simulink model "gtm_design"  (R2021b)
settings: Solver=VariableStepAuto  StartTime=0.0  StopTime=10.0  MinStep=0.00999  RelTol=1e-3
StopFcn:
  | MWSout=grabmws(bdroot);
  | MWSout.lastrun=datestr(now);
values from neighbouring files (symbols this model uses):
  knots2fps = 1.68781    [setup.m]
  s = tf('s')    [setup.m]
undefined symbols (not defined in the file or in its folder): Aero, aftfuel, aftfuel_pos, AILL, AILLC, AILR, AILRC, alpha_deg, alt0, altitude_ft, Ax_g, Ay_g, Az_g, b, beta_deg, bias, BRAKEC, Cbar, cg_pos0, cg_shift_gear, ControlMode, DamageCase, DamageModels, DamageOnsetTime, deltc, Earth, ELLIB, ELLIBC, ELLOB, ELLOBC, ELRIB, ELRIBC, ELROB, ELROBC, engl_ang, engl_pos, engr_ang, engr_pos, etas0, etas1, etasc_feedthrough, FLAPLC, FLAPLIB, FLAPLOB, FLAPRC, FLAPRIB, FLAPROB, FlightMode, FuelUsed_Init, fwdfuel, fwdfuel_pos, GEAR, GEARC, Inertia0, Inertia_shift_gear, Ixx_model, Iyy_model, Izz_model, KTAS, LandingGear ... (+66)
libraries: simulink_extras x98, LPVBlockLibrary x54, simulink_need_slupdate x30, aerolibconvert2 x27, simulink x7, aerolibtransform2 x6, uavalgslib x4, UserContent_lib x2, robotcorelib x1, uavutilslib x1
(part 4 of 9)

== system gtm_design/GTM_T2/Engines/Right_Engine Jetcat P70 ==
  Throttle : Inport
  pratio : Inport  Port=2
  tratio : Inport  Port=3
  BypassDynamics : Inport  Port=4
  qbar : Inport  Port=5
  S : Inport  Port=6
  Fuel Pump Voltage : Lookup  InputValues=fuelflow_table  Table=fuelpump_table  LookUpMeth=Interpolation-Use End Values
  Product2 : Product  RndMeth=Zero
  RPMref_2_EGT : Polyval  Coefs=Coeff_EGT
  RPMref_2_FuelFlow : Polyval  Coefs=Coeff_fuelflow
  RPMref_2_Thrust : Polyval  Coefs=Coeff_thrust
  Saturation : Saturate  UpperLimit=inf  LowerLimit=0
  Simple Ram Drag Model : MATLAB Function  TreatAsAtomicUnit=on
  Sum : Sum  Inputs=-+|
  Switch : Switch  Criteria=u2 ~= 0
  Terminator : Terminator
  Throttle Lag1 : Subsystem
  Throttle2 : InportShadow
  Throttle_2_RPMref : Polyval  Coefs=Coeff_throttle
  UnScale_Ref_RPM : Gain  Gain=123000/100
  angular momentum : Gain  Gain=(pi*shaft_dia^4/32) * shaft_len * density * (2*pi/60)
  Thrust (lbf) : Outport
  RPM : Outport  Port=2
  h (slg-ft^2/s) : Outport  Port=3
  Fuel Pump Voltage (V) : Outport  Port=4
  EGT (deg C) : Outport  Port=5
  Fuel Flow (lbs/min) : Outport  Port=6
  wires:
  Saturation/1 -> Thrust (lbf)/1
  Sum/1 -> Saturation/1
  Product2/1 -> Sum/2
  Simple Ram Drag Model/1(ram_drag) -> Sum/1
  S/1 -> Simple Ram Drag Model/2(S)
  qbar/1 -> Simple Ram Drag Model/1(qbar)
  Throttle2/1 -> Switch/1
  BypassDynamics/1 -> Switch/2
  Throttle Lag1/1(y) -> Switch/3  "Throttle_Lag"
  Switch/1 -> Throttle_2_RPMref/1
  Throttle/1 -> Throttle Lag1/1(throttle)
  Throttle_2_RPMref/1 -> RPMref_2_Thrust/1, UnScale_Ref_RPM/1, RPMref_2_EGT/1, RPMref_2_FuelFlow/1
  angular momentum/1 -> h (slg-ft^2/s)/1
  UnScale_Ref_RPM/1 -> angular momentum/1, RPM/1
  tratio/1 -> Terminator/1
  RPMref_2_Thrust/1 -> Product2/1
  RPMref_2_FuelFlow/1 -> Fuel Flow (lbs/min)/1, Fuel Pump Voltage/1
  pratio/1 -> Product2/2
  Fuel Pump Voltage/1 -> Fuel Pump Voltage (V)/1
  RPMref_2_EGT/1 -> EGT (deg C)/1

== system gtm_design/GTM_T2/Landing Gear/LandingGear ==
  cg : Inport  PortDimensions=3
  EulerAngles (Rad) : Inport  Port=2  PortDimensions=3
  Altitude (ft) : Inport  Port=3  PortDimensions=1
  pqr (Rad/sec) : Inport  Port=4  PortDimensions=3
  Vbody (ft/sec) : Inport  Port=5  PortDimensions=3
  Heading (Rad) : Inport  Port=6  PortDimensions=1
  Brake (0-1) : Inport  Port=7  PortDimensions=1
  Steer (deg) : Inport  Port=8  PortDimensions=1
  geardown (0/1) : Inport  Port=9  PortDimensions=1
  Data Type Conversion : DataTypeConversion  OutDataTypeStr=int32
  Euler to DCM1 : Subsystem
  Math Function : Math  Operator=transpose  SignedPower=on  SaturateOnIntegerOverflow=on
  Math Function1 : Math  Operator=transpose  SignedPower=on  SaturateOnIntegerOverflow=on
  Product : Product  Multiplication=Matrix(*)  RndMeth=Zero
  Reshape : Reshape
  S-Function1 : S-Function  FunctionName=gear_sfcn  SFunctionDeploymentMode=off  EnableBusSupport=off
  Subsystem : Subsystem
  Wheel Positions : Constant  Value=[NoseWheelPos(:);LeftMainPos(:); RightMainPos(:)];
  Wheel Positions1 : Constant  Value=SpringConst
  Wheel Positions2 : Constant  Value=DampingConst
  Wheel Positions3 : Constant  Value=MountStiffness
  Wheel Positions4 : Constant  Value=StrokeLength
  Wheel Positions5 : Constant  Value=MountDamping
  F_gear : Outport
  M_gear : Outport  Port=2
  Contact : Outport  Port=3
  wires:
  Wheel Positions5/1 -> S-Function1/5
  Math Function1/1 -> Product/1
  Vbody (ft/sec)/1 -> Product/2
  Euler to DCM1/1(DCM) -> Math Function1/1, Math Function/1
  Math Function/1 -> Reshape/1
  EulerAngles (Rad)/1 -> Euler to DCM1/1("Euler ")
  Altitude (ft)/1 -> Subsystem/1(Alt)
  geardown (0/1)/1 -> Data Type Conversion/1
  Wheel Positions/1 -> S-Function1/1
  Wheel Positions1/1 -> S-Function1/2
  Wheel Positions2/1 -> S-Function1/3
  Wheel Positions3/1 -> S-Function1/4
  Wheel Positions4/1 -> S-Function1/6
  cg/1 -> S-Function1/7
  Reshape/1 -> S-Function1/8
  Subsystem/1(cg_wrt_rwy) -> S-Function1/9
  pqr (Rad/sec)/1 -> S-Function1/10
  Product/1 -> S-Function1/11  "Vned"
  Heading (Rad)/1 -> S-Function1/12
  Brake (0-1)/1 -> S-Function1/13
  Steer (deg)/1 -> S-Function1/14
  Data Type Conversion/1 -> S-Function1/15
  S-Function1/1 -> F_gear/1
  S-Function1/2 -> M_gear/1
  S-Function1/3 -> Contact/1

== system gtm_design/GTM_T2/Sensors/Air Data ==
  EOM_State : Inport
  AuxVars : Inport  Port=2
  -50/+350 : Saturate  UpperLimit=350  LowerLimit=-50
  Bus Selector1 : BusSelector  OutputSignals=alpha,beta,qbar,tas,tratio
  Bus Selector2 : BusSelector  OutputSignals=altitude
  First Order Filter : Subsystem  mask(first order filter){tau=6}
      mask help:
      | __1__
      |  tau s+1
      |
      | First order filter  transfer function
      | with integrator IC = input  at time=0
      | If tau < Simulation Timestep, input is passed through unchanged
      | Simulation timestep must be a variable in the model/base workspace named
      | "Timestep"
      mask Help:
      | This block models a first order filter with the initial condition
      | on the integrator set to the steady state value for constant input.
      | time constant is an input
      mask Display: fprintf('  1\n--------------\n %2.1g s + 1', tau)
  Gain4 : Gain  Gain=59
  Sensor Model1 : Subsystem  mask(Sensor Model){noise_on=SensorNoise.On, sigma=SensorNoise.beta.Std, seed=878224, bias=SensorNoise.beta.Bias, scf=SensorNoise.beta.Scf}
      mask prompts: noise_on "on/off"; scf "scale factor:"
      mask help:
      | Add bias, scale factor, and white noise to a signal
      |
      | - 'on/off': 1 = noise on, 0 = noise off.
      | - 'sigma' : Standard deviation of white noise.
      | - 'seed'  : Random number seed. Generated numbers
      |   change between each simulation run, but the random number
      |   sequences do not change between Matlab sessions unless a
      |   new seed is specified.
      | - 'bias'  : Constant mean value offset of white noise.
      | - 'scale factor' : Scale factor applied to original signal.
      mask Display: disp('bias/scf/noise')
  Sensor Model2 : Subsystem  mask(Sensor Model){noise_on=SensorNoise.On, sigma=SensorNoise.KTAS.Std, seed=878654, bias=SensorNoise.KTAS.Bias, scf=SensorNoise.KTAS.Scf}
      mask prompts: noise_on "on/off"; scf "scale factor:"
      mask help:
      | Add bias, scale factor, and white noise to a signal
      |
      | - 'on/off': 1 = noise on, 0 = noise off.
      | - 'sigma' : Standard deviation of white noise.
      | - 'seed'  : Random number seed. Generated numbers
      |   change between each simulation run, but the random number
      |   sequences do not change between Matlab sessions unless a
      |   new seed is specified.
      | - 'bias'  : Constant mean value offset of white noise.
      | - 'scale factor' : Scale factor applied to original signal.
      mask Display: disp('bias/scf/noise')
  Sensor Model3 : Subsystem  mask(Sensor Model){noise_on=SensorNoise.On, sigma=SensorNoise.dyn_press.Std, seed=848234, bias=SensorNoise.dyn_press.Bias, scf=SensorNoise.dyn_press.Scf}
      mask prompts: noise_on "on/off"; scf "scale factor:"
      mask help:
      | Add bias, scale factor, and white noise to a signal
      |
      | - 'on/off': 1 = noise on, 0 = noise off.
      | - 'sigma' : Standard deviation of white noise.
      | - 'seed'  : Random number seed. Generated numbers
      |   change between each simulation run, but the random number
      |   sequences do not change between Matlab sessions unless a
      |   new seed is specified.
      | - 'bias'  : Constant mean value offset of white noise.
      | - 'scale factor' : Scale factor applied to original signal.
      mask Display: disp('bias/scf/noise')
  Sensor Model4 : Subsystem  mask(Sensor Model){noise_on=SensorNoise.On, sigma=SensorNoise.tempamb.Std, seed=878634, bias=SensorNoise.tempamb.Bias, scf=SensorNoise.tempamb.Scf}
      mask prompts: noise_on "on/off"; scf "scale factor:"
      mask help:
      | Add bias, scale factor, and white noise to a signal
      |
      | - 'on/off': 1 = noise on, 0 = noise off.
      | - 'sigma' : Standard deviation of white noise.
      | - 'seed'  : Random number seed. Generated numbers
      |   change between each simulation run, but the random number
      |   sequences do not change between Matlab sessions unless a
      |   new seed is specified.
      | - 'bias'  : Constant mean value offset of white noise.
      | - 'scale factor' : Scale factor applied to original signal.
      mask Display: disp('bias/scf/noise')
  Sensor Model5 : Subsystem  mask(Sensor Model){noise_on=SensorNoise.On, sigma=SensorNoise.alpha.Std, seed=278234, bias=SensorNoise.alpha.Bias, scf=SensorNoise.alpha.Scf}
      mask prompts: noise_on "on/off"; scf "scale factor:"
      mask help:
      | Add bias, scale factor, and white noise to a signal
      |
      | - 'on/off': 1 = noise on, 0 = noise off.
      | - 'sigma' : Standard deviation of white noise.
      | - 'seed'  : Random number seed. Generated numbers
      |   change between each simulation run, but the random number
      |   sequences do not change between Matlab sessions unless a
      |   new seed is specified.
      | - 'bias'  : Constant mean value offset of white noise.
      | - 'scale factor' : Scale factor applied to original signal.
      mask Display: disp('bias/scf/noise')
  Sensor Model6 : Subsystem  mask(Sensor Model){noise_on=SensorNoise.On, sigma=SensorNoise.baro_alt.Std, seed=878654, bias=SensorNoise.baro_alt.Bias, scf=SensorNoise.baro_alt.Scf}
      mask prompts: noise_on "on/off"; scf "scale factor:"
      mask help:
      | Add bias, scale factor, and white noise to a signal
      |
      | - 'on/off': 1 = noise on, 0 = noise off.
      | - 'sigma' : Standard deviation of white noise.
      | - 'seed'  : Random number seed. Generated numbers
      |   change between each simulation run, but the random number
      |   sequences do not change between Matlab sessions unless a
      |   new seed is specified.
      | - 'bias'  : Constant mean value offset of white noise.
      | - 'scale factor' : Scale factor applied to original signal.
      mask Display: disp('bias/scf/noise')
  pitot bus : BusCreator  Inputs=6
  AirData : Outport
  wires:
  Bus Selector1/5 -> First Order Filter/1(In)  "<tratio>"
  Sensor Model3/1(Out1) -> pitot bus/3  "qbar_psf"
  Bus Selector1/3 -> Sensor Model3/1(In1)  "<qbar>"
  pitot bus/1 -> AirData/1
  Gain4/1 -> Sensor Model4/1(In1)
  Sensor Model4/1(Out1) -> -50/+350/1
  -50/+350/1 -> pitot bus/5  "TEMPAMB_degF"
  First Order Filter/1(Out) -> Gain4/1
  Bus Selector1/1 -> Sensor Model5/1(In1)  "<alpha>"
  Bus Selector1/2 -> Sensor Model1/1(In1)  "<beta>"
  Sensor Model5/1(Out1) -> pitot bus/1  "alpha_deg"
  Sensor Model1/1(Out1) -> pitot bus/2  "beta_deg"
  Bus Selector1/4 -> Sensor Model2/1(In1)  "<tas>"
  Sensor Model2/1(Out1) -> pitot bus/4  "KTAS"
  AuxVars/1 -> Bus Selector1/1
  Bus Selector2/1 -> Sensor Model6/1(In1)  "<altitude>"
  Sensor Model6/1(Out1) -> pitot bus/6  "altitude_ft"
  EOM_State/1 -> Bus Selector2/1

== system gtm_design/GTM_T2/Sensors/Engine ECU 8 Hz ==
  Engines : Inport
  8 Hz : ZeroOrderHold  SampleTime=round(1/Timestep/8)*Timestep
  Bus Creator : BusCreator  Inputs=6
  Bus Selector : BusSelector  OutputSignals=RPML,PUMPVL,EGTL,RPMR,PUMPVR,EGTR
  RPM resolution : Quantizer  QuantizationInterval=500
      settings: AttributesFormatString=%<QuantizationInterval>
  RPM resolution1 : Quantizer  QuantizationInterval=500
      settings: AttributesFormatString=%<QuantizationInterval>
  RT : RateTransition
  Voltage resolution : Quantizer  QuantizationInterval=0.025
      settings: AttributesFormatString=%<QuantizationInterval>
  Voltage resolution1 : Quantizer  QuantizationInterval=0.025
      settings: AttributesFormatString=%<QuantizationInterval>
  deg C resolution : Quantizer  QuantizationInterval=4.6
      settings: AttributesFormatString=%<QuantizationInterval>
  deg C resolution1 : Quantizer  QuantizationInterval=4.6
      settings: AttributesFormatString=%<QuantizationInterval>
  ECU : Outport
  wires:
  8 Hz/1 -> RT/1
  Bus Creator/1 -> 8 Hz/1
  RT/1 -> ECU/1
  RPM resolution/1 -> Bus Creator/1  "RPML"
  Engines/1 -> Bus Selector/1
  deg C resolution/1 -> Bus Creator/3  "EGTL"
  RPM resolution1/1 -> Bus Creator/4  "RPMR"
  Bus Selector/1 -> RPM resolution/1  "<RPML>"
  Bus Selector/2 -> Voltage resolution/1  "<PUMPVL>"
  Bus Selector/3 -> deg C resolution/1  "<EGTL>"
  Bus Selector/4 -> RPM resolution1/1  "<RPMR>"
  Bus Selector/5 -> Voltage resolution1/1  "<PUMPVR>"
  Bus Selector/6 -> deg C resolution1/1  "<EGTR>"
  deg C resolution1/1 -> Bus Creator/6  "EGTR"
  Voltage resolution/1 -> Bus Creator/2  "PUMPVL"
  Voltage resolution1/1 -> Bus Creator/5  "PUMPVR"

== system gtm_design/GTM_T2/Sensors/MAG3 IMU ==
  AuxVars : Inport
  EOM_State : Inport  Port=2
  +/- 10g : Saturate  UpperLimit=10  LowerLimit=-10
  +/- 10g1 : Saturate  UpperLimit=10  LowerLimit=-10
  +/- 10g2 : Saturate  UpperLimit=10  LowerLimit=-10
  +/- 600 deg/sec : Saturate  UpperLimit=600  LowerLimit=-600
  +/- 600 deg/sec1 : Saturate  UpperLimit=600  LowerLimit=-600
  +/- 600 deg/sec2 : Saturate  UpperLimit=600  LowerLimit=-600
  Bus Selector2 : BusSelector  OutputSignals=Ax,Ay,Az
  Bus Selector3 : BusSelector  OutputSignals=pb,qb,rb
  MIDG bus : BusCreator  Inputs=6
  Radians to Degrees3 : simulink_extras/Transformations/Radians to Degrees
  Radians to Degrees4 : simulink_extras/Transformations/Radians to Degrees
  Radians to Degrees5 : simulink_extras/Transformations/Radians to Degrees
  Sensor Model1 : Subsystem  mask(Sensor Model){noise_on=SensorNoise.On, sigma=SensorNoise.MAG3.qdeg.Std, seed=871234, bias=SensorNoise.MAG3.qdeg.Bias, scf=SensorNoise.MAG3.qdeg.Scf}
      mask prompts: noise_on "on/off"; scf "scale factor:"
      mask help:
      | Add bias, scale factor, and white noise to a signal
      |
      | - 'on/off': 1 = noise on, 0 = noise off.
      | - 'sigma' : Standard deviation of white noise.
      | - 'seed'  : Random number seed. Generated numbers
      |   change between each simulation run, but the random number
      |   sequences do not change between Matlab sessions unless a
      |   new seed is specified.
      | - 'bias'  : Constant mean value offset of white noise.
      | - 'scale factor' : Scale factor applied to original signal.
      mask Display: disp('bias/scf/noise')
  Sensor Model2 : Subsystem  mask(Sensor Model){noise_on=SensorNoise.On, sigma=SensorNoise.MAG3.rdeg.Std, seed=878134, bias=SensorNoise.MAG3.rdeg.Bias, scf=SensorNoise.MAG3.rdeg.Scf}
      mask prompts: noise_on "on/off"; scf "scale factor:"
      mask help:
      | Add bias, scale factor, and white noise to a signal
      |
      | - 'on/off': 1 = noise on, 0 = noise off.
      | - 'sigma' : Standard deviation of white noise.
      | - 'seed'  : Random number seed. Generated numbers
      |   change between each simulation run, but the random number
      |   sequences do not change between Matlab sessions unless a
      |   new seed is specified.
      | - 'bias'  : Constant mean value offset of white noise.
      | - 'scale factor' : Scale factor applied to original signal.
      mask Display: disp('bias/scf/noise')
  Sensor Model3 : Subsystem  mask(Sensor Model){noise_on=SensorNoise.On, sigma=SensorNoise.MAG3.nxbody.Std, seed=878234, bias=SensorNoise.MAG3.nxbody.Bias, scf=SensorNoise.MAG3.nxbody.Scf}
      mask prompts: noise_on "on/off"; scf "scale factor:"
      mask help:
      | Add bias, scale factor, and white noise to a signal
      |
      | - 'on/off': 1 = noise on, 0 = noise off.
      | - 'sigma' : Standard deviation of white noise.
      | - 'seed'  : Random number seed. Generated numbers
      |   change between each simulation run, but the random number
      |   sequences do not change between Matlab sessions unless a
      |   new seed is specified.
      | - 'bias'  : Constant mean value offset of white noise.
      | - 'scale factor' : Scale factor applied to original signal.
      mask Display: disp('bias/scf/noise')
  Sensor Model4 : Subsystem  mask(Sensor Model){noise_on=SensorNoise.On, sigma=SensorNoise.MAG3.nybody.Std, seed=8782345, bias=SensorNoise.MAG3.nybody.Bias, scf=SensorNoise.MAG3.nybody.Scf}
      mask prompts: noise_on "on/off"; scf "scale factor:"
      mask help:
      | Add bias, scale factor, and white noise to a signal
      |
      | - 'on/off': 1 = noise on, 0 = noise off.
      | - 'sigma' : Standard deviation of white noise.
      | - 'seed'  : Random number seed. Generated numbers
      |   change between each simulation run, but the random number
      |   sequences do not change between Matlab sessions unless a
      |   new seed is specified.
      | - 'bias'  : Constant mean value offset of white noise.
      | - 'scale factor' : Scale factor applied to original signal.
      mask Display: disp('bias/scf/noise')
  Sensor Model5 : Subsystem  mask(Sensor Model){noise_on=SensorNoise.On, sigma=SensorNoise.MAG3.pdeg.Std, seed=878233, bias=SensorNoise.MAG3.pdeg.Bias, scf=SensorNoise.MAG3.pdeg.Scf}
      mask prompts: noise_on "on/off"; scf "scale factor:"
      mask help:
      | Add bias, scale factor, and white noise to a signal
      |
      | - 'on/off': 1 = noise on, 0 = noise off.
      | - 'sigma' : Standard deviation of white noise.
      | - 'seed'  : Random number seed. Generated numbers
      |   change between each simulation run, but the random number
      |   sequences do not change between Matlab sessions unless a
      |   new seed is specified.
      | - 'bias'  : Constant mean value offset of white noise.
      | - 'scale factor' : Scale factor applied to original signal.
      mask Display: disp('bias/scf/noise')
  Sensor Model6 : Subsystem  mask(Sensor Model){noise_on=SensorNoise.On, sigma=SensorNoise.MAG3.nzbody.Std, seed=878236, bias=SensorNoise.MAG3.nzbody.Bias, scf=SensorNoise.MAG3.nzbody.Scf}
      mask prompts: noise_on "on/off"; scf "scale factor:"
      mask help:
      | Add bias, scale factor, and white noise to a signal
      |
      | - 'on/off': 1 = noise on, 0 = noise off.
      | - 'sigma' : Standard deviation of white noise.
      | - 'seed'  : Random number seed. Generated numbers
      |   change between each simulation run, but the random number
      |   sequences do not change between Matlab sessions unless a
      |   new seed is specified.
      | - 'bias'  : Constant mean value offset of white noise.
      | - 'scale factor' : Scale factor applied to original signal.
      mask Display: disp('bias/scf/noise')
  MAG3 : Outport
  wires:
  +/- 10g2/1 -> MIDG bus/6  "Az_g"
  +/- 10g1/1 -> MIDG bus/5  "Ay_g"
  +/- 10g/1 -> MIDG bus/4  "Ax_g"
  +/- 600 deg/sec2/1 -> MIDG bus/3  "r_deg"
  +/- 600 deg/sec1/1 -> MIDG bus/2  "q_deg"
  +/- 600 deg/sec/1 -> MIDG bus/1  "p_deg"
  EOM_State/1 -> Bus Selector3/1
  Bus Selector3/1 -> Radians to Degrees3/1  "<pb>"
  Bus Selector3/2 -> Radians to Degrees4/1  "<qb>"
  Bus Selector3/3 -> Radians to Degrees5/1  "<rb>"
  Bus Selector2/1 -> Sensor Model3/1(In1)  "<Ax>"
  Bus Selector2/2 -> Sensor Model4/1(In1)  "<Ay>"
  Bus Selector2/3 -> Sensor Model6/1(In1)  "<Az>"
  Radians to Degrees3/1 -> Sensor Model5/1(In1)
  Radians to Degrees4/1 -> Sensor Model1/1(In1)
  Radians to Degrees5/1 -> Sensor Model2/1(In1)
  Sensor Model1/1(Out1) -> +/- 600 deg/sec1/1
  Sensor Model2/1(Out1) -> +/- 600 deg/sec2/1
  Sensor Model3/1(Out1) -> +/- 10g/1
  Sensor Model4/1(Out1) -> +/- 10g1/1
  Sensor Model6/1(Out1) -> +/- 10g2/1
  Sensor Model5/1(Out1) -> +/- 600 deg/sec/1
  AuxVars/1 -> Bus Selector2/1
  MIDG bus/1 -> MAG3/1

== system gtm_design/GTM_T2/Sensors/MIDG II 50 Hz ==
  AuxVars : Inport
  EOM_State : Inport  Port=2
  0.01 deg Resolution : Quantizer  QuantizationInterval=0.01
  0.01 deg Resolution1 : Quantizer  QuantizationInterval=0.01
  0.01 deg Resolution2 : Quantizer  QuantizationInterval=0.01
  0.01 m Resolution1 : Quantizer  QuantizationInterval=0.01
  0.01 m/s Resolution : Quantizer  QuantizationInterval=0.01
  0.01 m/s Resolution1 : Quantizer  QuantizationInterval=0.01
  0.01 m/s Resolution2 : Quantizer  QuantizationInterval=0.01
  1e-7 deg Resolution2 : Quantizer  QuantizationInterval=1e-7
  1e-7 deg Resolution3 : Quantizer  QuantizationInterval=1e-7
  Bus Selector3 : BusSelector  OutputSignals=phi,theta,psi,latitude,longitude,altitude
  Bus Selector8 : BusSelector  OutputSignals=Vn,Ve,Vd
  Bus to Vector : BusToVector
  Gain10 : Gain  Gain=0.5144
  Gain11 : Gain  Gain=-0.5144
  Gain12 : Gain  Gain=0.3048
  Gain{13..17} (5 alike) : Gain  Gain=180/pi
  Gain9 : Gain  Gain=0.5144
  MIDG Labels : Subsystem
  MIDG bus : BusCreator  Inputs=9
  Map+/-180 : Subsystem
  Rate Transition : RateTransition  InitialCondition=[StatesInp(10:11)*180/pi;0;StatesInp(7)*180/pi;StatesInp(8)*180/pi;StatesInp(9)*0.3048;StatesInp(1)*0.3048*cos(StatesInp(11))+StatesInp(3)*0.3048*sin(StatesInp(11));0;-StatesInp(1)*0.3048*sin(StatesInp(11))+StatesInp(3)*0.3048*cos(StatesInp(11))]
  Sensor Model7 : Subsystem  mask(Sensor Model){noise_on=SensorNoise.On, sigma=SensorNoise.MIDG.psi.Std, seed=878232, bias=SensorNoise.MIDG.psi.Bias, scf=SensorNoise.MIDG.psi.Scf}
      mask prompts: noise_on "on/off"; scf "scale factor:"
      mask help:
      | Add bias, scale factor, and white noise to a signal
      |
      | - 'on/off': 1 = noise on, 0 = noise off.
      | - 'sigma' : Standard deviation of white noise.
      | - 'seed'  : Random number seed. Generated numbers
      |   change between each simulation run, but the random number
      |   sequences do not change between Matlab sessions unless a
      |   new seed is specified.
      | - 'bias'  : Constant mean value offset of white noise.
      | - 'scale factor' : Scale factor applied to original signal.
      mask Display: disp('bias/scf/noise')
  Sensor Model8 : Subsystem  mask(Sensor Model){noise_on=SensorNoise.On, sigma=SensorNoise.MIDG.theta.Std, seed=878231, bias=SensorNoise.MIDG.theta.Bias, scf=SensorNoise.MIDG.theta.Scf}
      mask prompts: noise_on "on/off"; scf "scale factor:"
      mask help:
      | Add bias, scale factor, and white noise to a signal
      |
      | - 'on/off': 1 = noise on, 0 = noise off.
      | - 'sigma' : Standard deviation of white noise.
      | - 'seed'  : Random number seed. Generated numbers
      |   change between each simulation run, but the random number
      |   sequences do not change between Matlab sessions unless a
      |   new seed is specified.
      | - 'bias'  : Constant mean value offset of white noise.
      | - 'scale factor' : Scale factor applied to original signal.
      mask Display: disp('bias/scf/noise')
  Sensor Model9 : Subsystem  mask(Sensor Model){noise_on=SensorNoise.On, sigma=SensorNoise.MIDG.phi.Std, seed=878230, bias=SensorNoise.MIDG.phi.Bias, scf=SensorNoise.MIDG.phi.Scf}
      mask prompts: noise_on "on/off"; scf "scale factor:"
      mask help:
      | Add bias, scale factor, and white noise to a signal
      |
      | - 'on/off': 1 = noise on, 0 = noise off.
      | - 'sigma' : Standard deviation of white noise.
      | - 'seed'  : Random number seed. Generated numbers
      |   change between each simulation run, but the random number
      |   sequences do not change between Matlab sessions unless a
      |   new seed is specified.
      | - 'bias'  : Constant mean value offset of white noise.
      | - 'scale factor' : Scale factor applied to original signal.
      mask Display: disp('bias/scf/noise')
  TimeDelay with IC feedthrough : Subsystem  mask{TimeDelay=40e-3}
      mask prompts: TimeDelay "Time Delay (sec)"
      mask help:
      | Implements Continuous Time Transport Delay with initial
      | outputs set to feedthrough with no delay.
      |
      |   output = input;   for t<TimeDelay
      |   output = input(t-tdelay); for t>=TimeDelay
  Zero-Order Hold : ZeroOrderHold  SampleTime=round(1/Timestep/50)*Timestep
  MIDG : Outport
  wires:
  Bus to Vector/1 -> TimeDelay with IC feedthrough/1(I)
  TimeDelay with IC feedthrough/1(O) -> Zero-Order Hold/1
  MIDG bus/1 -> Bus to Vector/1
  Zero-Order Hold/1 -> Rate Transition/1
  EOM_State/1 -> Bus Selector3/1
  Bus Selector3/1 -> Gain13/1  "<phi>"
  Bus Selector3/2 -> Gain14/1  "<theta>"
  Bus Selector3/3 -> Gain15/1  "<psi>"
  Sensor Model7/1(Out1) -> 0.01 deg Resolution2/1
  Sensor Model8/1(Out1) -> 0.01 deg Resolution1/1
  Sensor Model9/1(Out1) -> 0.01 deg Resolution/1
  0.01 deg Resolution/1 -> MIDG bus/1  "phi"
  0.01 deg Resolution1/1 -> MIDG bus/2  "theta"
  0.01 deg Resolution2/1 -> Map+/-180/1(I)  "psi"
  1e-7 deg Resolution2/1 -> MIDG bus/4  "latitude"
  1e-7 deg Resolution3/1 -> MIDG bus/5  "longitude"
  Gain9/1 -> 0.01 m/s Resolution/1
  Gain10/1 -> 0.01 m/s Resolution1/1
  Gain11/1 -> 0.01 m/s Resolution2/1
  Gain12/1 -> 0.01 m Resolution1/1
  0.01 m/s Resolution/1 -> MIDG bus/7  "Vn"
  0.01 m/s Resolution1/1 -> MIDG bus/8  "Ve"
  Gain13/1 -> Sensor Model9/1(In1)
  Gain14/1 -> Sensor Model8/1(In1)
  Gain15/1 -> Sensor Model7/1(In1)
  Gain16/1 -> 1e-7 deg Resolution2/1
  Gain17/1 -> 1e-7 deg Resolution3/1
  Bus Selector8/1 -> Gain9/1  "<Vn>"
  Bus Selector8/2 -> Gain10/1  "<Ve>"
  Bus Selector8/3 -> Gain11/1  "<Vd>"
  Bus Selector3/4 -> Gain16/1  "<latitude>"
  Bus Selector3/5 -> Gain17/1  "<longitude>"
  Bus Selector3/6 -> Gain12/1  "<altitude>"
  AuxVars/1 -> Bus Selector8/1
  Map+/-180/1(O) -> MIDG bus/3  "psi"
  MIDG Labels/1(O) -> MIDG/1
  0.01 m/s Resolution2/1 -> MIDG bus/9  "Vu"
  Rate Transition/1 -> MIDG Labels/1(I)
  0.01 m Resolution1/1 -> MIDG bus/6  "altitude"

== system gtm_design/GTM_T2/Sensors/Surface Pots ==
  SurfacePos : Inport
  Bus Selector : BusSelector  OutputSignals=ELLOB,ELLIB,ELROB,ELRIB,AILL,AILR,RUDU,RUDL,FLAPLIB,FLAPLOB,FLAPRIB,FLAPROB  OutputAsBus=on
  Sensor Model5 : Subsystem  mask(Sensor Model){noise_on=SensorNoise.On, sigma=SensorNoise.pots.Std, seed=878239, bias=SensorNoise.pots.Bias, scf=SensorNoise.pots.Scf}
      mask prompts: noise_on "on/off"; scf "scale factor:"
      mask help:
      | Add bias, scale factor, and white noise to a signal
      |
      | - 'on/off': 1 = noise on, 0 = noise off.
      | - 'sigma' : Standard deviation of white noise.
      | - 'seed'  : Random number seed. Generated numbers
      |   change between each simulation run, but the random number
      |   sequences do not change between Matlab sessions unless a
      |   new seed is specified.
      | - 'bias'  : Constant mean value offset of white noise.
      | - 'scale factor' : Scale factor applied to original signal.
      mask Display: disp('bias/scf/noise')
  Surface Labels : Subsystem
  Pots : Outport
  wires:
  Bus Selector/1 -> Sensor Model5/1(In1)
  SurfacePos/1 -> Bus Selector/1
  Sensor Model5/1(Out1) -> Surface Labels/1(I)
  Surface Labels/1(O) -> Pots/1

== system gtm_design/GTM_T2/TransportDelay/AntiAliasing ==
  I : Inport
  Bus Assignment : BusAssignment  AssignedSignals=AirData.alpha_deg,AirData.beta_deg,AirData.qbar_psf,AirData.KTAS,AirData.TEMPAMB_degF,AirData.altitude_ft,MAG3.p_deg,MAG3.q_deg,MAG3.r_deg,MAG3.Ax_g,MAG3.Ay_g,MAG3.Az_g,SurfacePos.ELLOB,SurfacePos.ELLIB,SurfacePos.ELROB,SurfacePos.ELRIB,SurfacePos.AILL,SurfacePos.AILR,SurfacePos.RUDU,SurfacePos.RUDL,SurfacePos.FLAPLIB,SurfacePos.FLAPLOB,SurfacePos.FLAPRIB,SurfacePos.FLAPROB
  Bus Selector : BusSelector  OutputSignals=AirData.alpha_deg,AirData.beta_deg,AirData.qbar_psf,AirData.KTAS,AirData.TEMPAMB_degF,AirData.altitude_ft,MAG3.p_deg,MAG3.q_deg,MAG3.r_deg,MAG3.Ax_g,MAG3.Ay_g,MAG3.Az_g,SurfacePos.ELLOB,SurfacePos.ELLIB,SurfacePos.ELROB,SurfacePos.ELRIB,SurfacePos.AILL,SurfacePos.AILR,SurfacePos.RUDU,SurfacePos.RUDL,SurfacePos.FLAPLIB,SurfacePos.FLAPLOB,SurfacePos.FLAPRIB,SurfacePos.FLAPROB  OutputAsBus=on
  Bus to Vector : BusToVector
  Demux : Demux  Outputs=24
  First Order Filter Continuous : Subsystem  mask(first order filter){tau=1/2/pi/16}
      mask help:
      | __1__
      |  tau s+1
      |
      | First order filter  transfer function
      | with integrator IC = input  at time=0
      |
      | Uses continuous time integrator.
      mask Display: fprintf('  1\n--------------\n %2.1g s + 1', tau)
  O : Outport
  wires:
  Bus to Vector/1 -> First Order Filter Continuous/1(In)
  I/1 -> Bus Selector/1, Bus Assignment/1
  Bus Selector/1 -> Bus to Vector/1
  First Order Filter Continuous/1(Out) -> Demux/1
  Bus Assignment/1 -> O/1
  Demux/1 -> Bus Assignment/2
  Demux/2 -> Bus Assignment/3
  Demux/3 -> Bus Assignment/4
  Demux/4 -> Bus Assignment/5
  Demux/5 -> Bus Assignment/6
  Demux/6 -> Bus Assignment/7
  Demux/7 -> Bus Assignment/8
  Demux/8 -> Bus Assignment/9
  Demux/9 -> Bus Assignment/10
  Demux/10 -> Bus Assignment/11
  Demux/11 -> Bus Assignment/12
  Demux/12 -> Bus Assignment/13
  Demux/13 -> Bus Assignment/14
  Demux/14 -> Bus Assignment/15
  Demux/15 -> Bus Assignment/16
  Demux/16 -> Bus Assignment/17
  Demux/17 -> Bus Assignment/18
  Demux/18 -> Bus Assignment/19
  Demux/19 -> Bus Assignment/20
  Demux/20 -> Bus Assignment/21
  Demux/21 -> Bus Assignment/22
  Demux/22 -> Bus Assignment/23
  Demux/23 -> Bus Assignment/24
  Demux/24 -> Bus Assignment/25

== system gtm_design/GTM_T2/TransportDelay/Transport Delay on Bus ==
  In : Inport
  Bus Creator : BusCreator  Inputs=5
  Bus Selector : BusSelector  OutputSignals=AirData,MIDG,MAG3,SurfacePos,Engines
  BusDelay : Subsystem
  BusDelay1 : Subsystem
  BusDelay2 : Subsystem
  BusDelay3 : Subsystem
  BusDelay4 : Subsystem
  Out : Outport
  wires:
  In/1 -> Bus Selector/1
  Bus Selector/1 -> BusDelay/1(In1)  "<AirData>"
  Bus Selector/2 -> BusDelay1/1(In1)  "<MIDG>"
  Bus Selector/3 -> BusDelay2/1(In1)  "<MAG3>"
  Bus Selector/4 -> BusDelay3/1(In1)  "<SurfacePos>"
  Bus Selector/5 -> BusDelay4/1(In1)  "<Engines>"
  BusDelay/1(Out1) -> Bus Creator/1  "AirData"
  BusDelay1/1(Out1) -> Bus Creator/2  "MIDG"
  BusDelay2/1(Out1) -> Bus Creator/3  "MAG3"
  BusDelay3/1(Out1) -> Bus Creator/4  "SurfacePos"
  BusDelay4/1(Out1) -> Bus Creator/5  "Engines"
  Bus Creator/1 -> Out/1

== system gtm_design/GTM_T2/TransportDelay/Transport Delay on Bus1 ==
  In : Inport
  BusDelay : Subsystem
  Out : Outport
  wires:
  In/1 -> BusDelay/1(In1)
  BusDelay/1(Out1) -> Out/1

== system gtm_design/Guidance/Autopilot Step/Airspeed Step Command ==
  Action Port : ActionPort  ActionPortLabel=case [ 1 ]:
  Bus Creator1 : BusCreator  Inputs=7
  Constant : Constant  Value=alt0
  Constant2 : Constant  Value=0
  Constant3 : Constant  Value=0
  Constant4 : Constant  Value=0
  Constant5 : Constant  Value=etas0
  Constant6 : Constant
  Step : Step  Before=tas0  After=tas0+5  SampleTime=0
  cmd : Outport
  wires:
  Constant5/1 -> Bus Creator1/7  "etas_c_percent"
  Constant4/1 -> Bus Creator1/6  "p_c_deg"
  Constant/1 -> Bus Creator1/2  "alt_c_ft"
  Bus Creator1/1 -> cmd/1
  Constant2/1 -> Bus Creator1/4  "phi_c_deg"
  Constant6/1 -> Bus Creator1/5  "an_c_g"
  Constant3/1 -> Bus Creator1/3  "bet_c_deg"
  Step/1 -> Bus Creator1/1  "tas_c_knot"

== system gtm_design/Guidance/Autopilot Step/Altitude Step Command ==
  Action Port : ActionPort  ActionPortLabel=case [ 2 ]:
  Bus Creator1 : BusCreator  Inputs=7
  Constant1 : Constant  Value=tas0
  Constant2 : Constant  Value=0
  Constant3 : Constant  Value=0
  Constant4 : Constant  Value=0
  Constant5 : Constant  Value=etas0
  Constant6 : Constant
  Step : Step  Before=alt0  After=alt0+10  SampleTime=0
  cmd : Outport
  wires:
  Constant5/1 -> Bus Creator1/7  "etas_c_percent"
  Constant4/1 -> Bus Creator1/6  "p_c_deg"
  Step/1 -> Bus Creator1/2  "alt_c_ft"
  Bus Creator1/1 -> cmd/1
  Constant2/1 -> Bus Creator1/4  "phi_c_deg"
  Constant6/1 -> Bus Creator1/5  "an_c_g"
  Constant3/1 -> Bus Creator1/3  "bet_c_deg"
  Constant1/1 -> Bus Creator1/1  "tas_c_knot"

== system gtm_design/Guidance/Autopilot Step/Label ==
  I : Inport
  Bus Creator1 : BusCreator  Inputs=7
  Demux1 : Demux  Outputs=7
  O : Outport
  wires:
  Bus Creator1/1 -> O/1
  Demux1/4 -> Bus Creator1/4  "phi_c_deg"
  Demux1/2 -> Bus Creator1/2  "alt_c_ft"
  Demux1/6 -> Bus Creator1/6  "p_c_deg"
  Demux1/1 -> Bus Creator1/1  "tas_c_knot"
  Demux1/3 -> Bus Creator1/3  "bet_c_deg"
  Demux1/5 -> Bus Creator1/5  "an_c_g"
  Demux1/7 -> Bus Creator1/7  "etas_c_percent"
  I/1 -> Demux1/1

== system gtm_design/Guidance/Autopilot Step/Roll Angle Step Command ==
  Action Port : ActionPort  ActionPortLabel=case [ 4 ]:
  20deg @ 1sec : Step  After=30  SampleTime=0
  Bus Creator1 : BusCreator  Inputs=7
  Constant : Constant  Value=alt0
  Constant1 : Constant  Value=tas0
  Constant3 : Constant  Value=0
  Constant4 : Constant
  Constant5 : Constant  Value=etas0
  Constant6 : Constant  Value=0
  cmd : Outport
  wires:
  Constant1/1 -> Bus Creator1/1  "tas_c_knot"
  Constant3/1 -> Bus Creator1/3  "bet_c_deg"
  Constant4/1 -> Bus Creator1/5  "an_c_g"
  20deg @ 1sec/1 -> Bus Creator1/4  "phi_c_deg"
  Bus Creator1/1 -> cmd/1
  Constant/1 -> Bus Creator1/2  "alt_c_ft"
  Constant6/1 -> Bus Creator1/6  "p_c_deg"
  Constant5/1 -> Bus Creator1/7  "etas_c_percent"

== system gtm_design/Guidance/Autopilot Step/Sideslip Step Command ==
  Action Port : ActionPort  ActionPortLabel=case [ 3 ]:
  3deg @ 1sec : Step  After=3  SampleTime=0
  Bus Creator1 : BusCreator  Inputs=7
  Constant : Constant  Value=alt0
  Constant1 : Constant  Value=tas0
  Constant2 : Constant  Value=0
  Constant3 : Constant
  Constant4 : Constant  Value=0
  Constant5 : Constant  Value=etas0
  cmd : Outport
  wires:
  Constant1/1 -> Bus Creator1/1  "tas_c_knot"
  3deg @ 1sec/1 -> Bus Creator1/3  "bet_c_deg"
  Constant3/1 -> Bus Creator1/5  "an_c_g"
  Constant2/1 -> Bus Creator1/4  "phi_c_deg"
  Bus Creator1/1 -> cmd/1
  Constant/1 -> Bus Creator1/2  "alt_c_ft"
  Constant4/1 -> Bus Creator1/6  "p_c_deg"
  Constant5/1 -> Bus Creator1/7  "etas_c_percent"

== system gtm_design/Guidance/Autopilot Step/Zero ==
  Action Port : ActionPort  ActionPortLabel=default:
  Bus Creator1 : BusCreator  Inputs=7
  Constant : Constant  Value=alt0
  Constant1 : Constant  Value=tas0
  Constant2 : Constant  Value=0
  Constant3 : Constant  Value=0
  Constant4 : Constant
  Constant5 : Constant  Value=etas0
  Constant6 : Constant  Value=0
  cmd : Outport
  wires:
  Constant1/1 -> Bus Creator1/1  "tas_c_knot"
  Constant3/1 -> Bus Creator1/3  "bet_c_deg"
  Constant4/1 -> Bus Creator1/5  "an_c_g"
  Constant2/1 -> Bus Creator1/4  "phi_c_deg"
  Bus Creator1/1 -> cmd/1
  Constant/1 -> Bus Creator1/2  "alt_c_ft"
  Constant6/1 -> Bus Creator1/6  "p_c_deg"
  Constant5/1 -> Bus Creator1/7  "etas_c_percent"

== system gtm_design/Guidance/Autopilot Trajectory Tracking/Label ==
  I : Inport
  Bus Creator1 : BusCreator  Inputs=11
  Demux1 : Demux  Outputs=11
  O : Outport
  wires:
  Bus Creator1/1 -> O/1
  Demux1/4 -> Bus Creator1/4  "phi_c_deg"
  Demux1/2 -> Bus Creator1/2  "alt_c_ft"
  Demux1/6 -> Bus Creator1/6  "p_c_deg"
  Demux1/1 -> Bus Creator1/1  "tas_c_knot"
  Demux1/3 -> Bus Creator1/3  "bet_c_deg"
  Demux1/5 -> Bus Creator1/5  "an_c_g"
  Demux1/7 -> Bus Creator1/7  "etas_c_percent"
  I/1 -> Demux1/1
  Demux1/8 -> Bus Creator1/8
  Demux1/9 -> Bus Creator1/9
  Demux1/10 -> Bus Creator1/10
  Demux1/11 -> [DesiredCourse], Bus Creator1/11

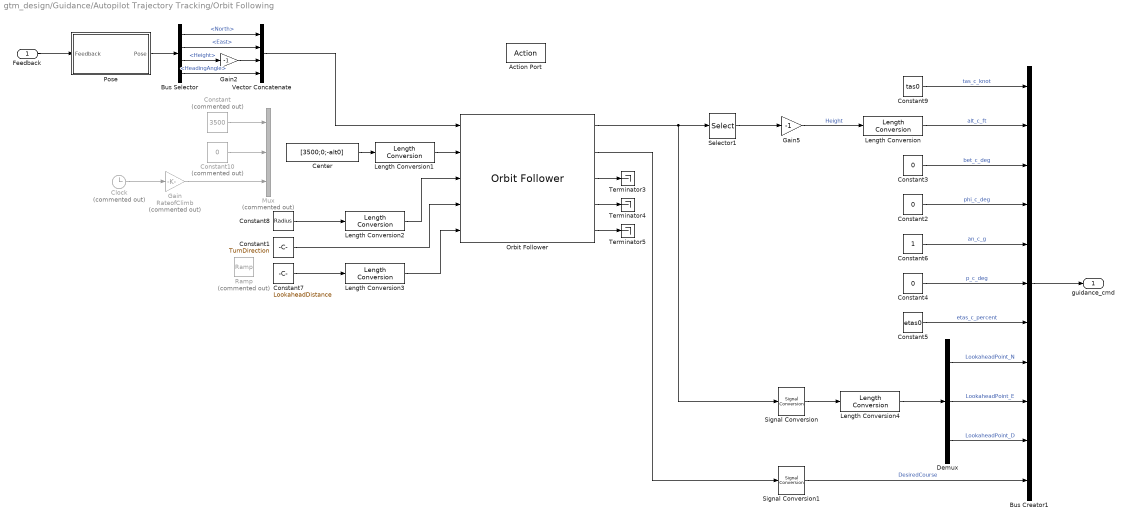
== system gtm_design/Guidance/Autopilot Trajectory Tracking/Orbit Following ==
  Feedback : Inport
  Action Port : ActionPort  ActionPortLabel=case [ 2 ]:
  Bus Creator1 : BusCreator  Inputs=11
  Bus Selector : BusSelector  OutputSignals=North,East,Height,HeadingAngle
  Center : Constant  Value=[3500;0;-alt0]  VectorParams1D=off
  Clock : Clock  Commented=on
  Constant : Constant  Commented=on  Value=3500
  Constant1 : Constant  Value=TurnDirection
  Constant10 : Constant  Commented=on  Value=0
  Constant2 : Constant  Value=0
  Constant3 : Constant  Value=0
  Constant4 : Constant  Value=0
  Constant5 : Constant  Value=etas0
  Constant6 : Constant
  Constant7 : Constant  Value=LookaheadDistance
  Constant8 : Constant  Value=Radius
  Constant9 : Constant  Value=tas0
  Demux : Demux  Outputs=3
  Gain : Gain  Commented=on  Gain=RateofClimb
  Gain2 : Gain  Gain=-1
  Gain5 : Gain  Gain=-1
  Length Conversion : aerolibconvert2/Length Conversion  IU=m  OU=ft
  Length Conversion1 : aerolibconvert2/Length Conversion  IU=ft  OU=m
  Length Conversion2 : aerolibconvert2/Length Conversion  IU=ft  OU=m
  Length Conversion3 : aerolibconvert2/Length Conversion  IU=ft  OU=m
  Length Conversion4 : aerolibconvert2/Length Conversion  IU=m  OU=ft
  Mux : Mux  Commented=on  Inputs=3
  Orbit Follower : uavalgslib/Orbit Follower  UAVType=fixed-wing  MinOrbitRadius=1  MinLookaheadDistance=0.1  ExternalReset=none  ShowCrossTrackErrorOutput=off  ShowNumTurnsOutput=off  SimulateUsing=Interpreted execution
      settings: SourceProductBaseCode=UV
  Pose : Subsystem
  Ramp : simulink/Sources/Ramp  Commented=on  slope=4  start=0  InitialOutput=2000
  Selector1 : Selector  InputPortWidth=3  IndexOptions=Index vector (dialog)  Indices=[3]  OutputSizes=1
  Signal Conversion : SignalConversion  OverrideOpt=off
  Signal Conversion1 : SignalConversion  OverrideOpt=off
  Terminator3 : Terminator
  Terminator4 : Terminator
  Terminator5 : Terminator
  Vector Concatenate : Concatenate  NumInputs=4
  guidance_cmd : Outport
  wires:
  Demux/1 -> Bus Creator1/8  "LookaheadPoint_N"
  Demux/2 -> Bus Creator1/9  "LookaheadPoint_E"
  Demux/3 -> Bus Creator1/10  "LookaheadPoint_D"
  Bus Selector/4 -> Vector Concatenate/4  "<HeadingAngle>"
  Pose/1(Pose) -> Bus Selector/1
  Selector1/1 -> Gain5/1
  Feedback/1 -> Pose/1(Feedback)
  Vector Concatenate/1 -> Orbit Follower/1
  Bus Selector/2 -> Vector Concatenate/2  "<East>"
  Orbit Follower/2 -> Signal Conversion1/1
  Bus Selector/3 -> Gain2/1  "<Height>"
  Gain2/1 -> Vector Concatenate/3
  Orbit Follower/1 -> Selector1/1, Signal Conversion/1
  Bus Selector/1 -> Vector Concatenate/1  "<North>"
  Gain5/1 -> Length Conversion/1  "Height"
  Constant9/1 -> Bus Creator1/1  "tas_c_knot"
  Constant3/1 -> Bus Creator1/3  "bet_c_deg"
  Constant6/1 -> Bus Creator1/5  "an_c_g"
  Constant2/1 -> Bus Creator1/4  "phi_c_deg"
  Bus Creator1/1 -> guidance_cmd/1
  Constant4/1 -> Bus Creator1/6  "p_c_deg"
  Constant5/1 -> Bus Creator1/7  "etas_c_percent"
  Constant7/1 -> Length Conversion3/1
  Orbit Follower/3 -> Terminator3/1
  Constant1/1 -> Orbit Follower/4
  Orbit Follower/5 -> Terminator5/1
  Constant8/1 -> Length Conversion2/1
  Orbit Follower/4 -> Terminator4/1
  Signal Conversion/1 -> Length Conversion4/1
  Signal Conversion1/1 -> Bus Creator1/11  "DesiredCourse"
  Length Conversion1/1 -> Orbit Follower/2
  Length Conversion2/1 -> Orbit Follower/3
  Length Conversion3/1 -> Orbit Follower/5
  Length Conversion4/1 -> Demux/1
  Length Conversion/1 -> Bus Creator1/2  "alt_c_ft"
  Constant/1 -> Mux/1
  Constant10/1 -> Mux/2
  Clock/1 -> Gain/1
  Gain/1 -> Mux/3
  Center/1 -> Length Conversion1/1

== system gtm_design/Guidance/Autopilot Trajectory Tracking/Waypoint Following ==
  Feedback : Inport
  Action Port : ActionPort  ActionPortLabel=case [ 1 ]:
  Bus Creator1 : BusCreator  Inputs=11
  Bus Selector : BusSelector  OutputSignals=North,East,Height,HeadingAngle
  Constant1 : Constant  Value=tas0
  Constant2 : Constant  Value=0
  Constant3 : Constant  Value=0
  Constant4 : Constant  Value=0
  Constant5 : Constant  Value=etas0
  Constant6 : Constant
  Constant9 : Constant  Value=LookaheadDistance
  Demux : Demux  Outputs=3
  Display : Display
  Display1 : Display
  Gain2 : Gain  Gain=-1
  Gain5 : Gain  Gain=-1
  Length Conversion : aerolibconvert2/Length Conversion  IU=m  OU=ft
  Length Conversion1 : aerolibconvert2/Length Conversion  IU=ft  OU=m
  Length Conversion2 : aerolibconvert2/Length Conversion  IU=ft  OU=m
  Length Conversion4 : aerolibconvert2/Length Conversion  IU=m  OU=ft
  Pose : Subsystem
  Selector1 : Selector  InputPortWidth=3  IndexOptions=Index vector (dialog)  Indices=[3]  OutputSizes=1
  Signal Conversion : SignalConversion  OverrideOpt=off
  Signal Conversion1 : SignalConversion  OverrideOpt=off
  Terminator3 : Terminator
  Terminator4 : Terminator
  Vector Concatenate : Concatenate  NumInputs=4
  Waypoint Follower : uavalgslib/Waypoint Follower  UAVType=fixed-wing  StartFrom=first  TransitionRadiusSource=internal  TransitionRadius=TransitionRadius  MinLookaheadDistance=0.1  YawInput=off  ShowCrossTrackErrorOutput=off  ShowStatusOutput=off  SimulateUsing=Interpreted execution
      settings: SourceProductBaseCode=UV
  Waypoints : Constant  Value=Waypoints  VectorParams1D=off
  guidance_cmd : Outport
  wires:
  Constant5/1 -> Bus Creator1/7  "etas_c_percent"
  Constant4/1 -> Bus Creator1/6  "p_c_deg"
  Bus Creator1/1 -> guidance_cmd/1
  Constant2/1 -> Bus Creator1/4  "phi_c_deg"
  Constant6/1 -> Bus Creator1/5  "an_c_g"
  Constant3/1 -> Bus Creator1/3  "bet_c_deg"
  Constant1/1 -> Bus Creator1/1  "tas_c_knot"
  Gain5/1 -> Length Conversion/1  "Height"
  Bus Selector/1 -> Vector Concatenate/1  "<North>"
  Waypoint Follower/1 -> Display/1, Selector1/1, Signal Conversion/1  "LookaheadPoint"
  Gain2/1 -> Vector Concatenate/3
  Bus Selector/3 -> Gain2/1  "<Height>"
  Waypoint Follower/4 -> Terminator4/1
  Bus Selector/2 -> Vector Concatenate/2  "<East>"
  Vector Concatenate/1 -> Waypoint Follower/1
  Feedback/1 -> Pose/1(Feedback)
  Waypoints/1 -> Length Conversion1/1
  Selector1/1 -> Gain5/1
  Constant9/1 -> Length Conversion2/1
  Pose/1(Pose) -> Bus Selector/1
  Bus Selector/4 -> Vector Concatenate/4  "<HeadingAngle>"
  Length Conversion/1 -> Bus Creator1/2  "alt_c_ft"
  Waypoint Follower/3 -> Terminator3/1
  Demux/3 -> Bus Creator1/10  "LookaheadPoint_D"
  Demux/2 -> Bus Creator1/9  "LookaheadPoint_E"
  Demux/1 -> Bus Creator1/8  "LookaheadPoint_N"
  Signal Conversion/1 -> Length Conversion4/1  "LookaheadPoint"
  Signal Conversion1/1 -> Display1/1, Bus Creator1/11  "DesiredCourse"
  Waypoint Follower/2 -> Signal Conversion1/1  "DesiredCourse"
  Length Conversion1/1 -> Waypoint Follower/2
  Length Conversion2/1 -> Waypoint Follower/3
  Length Conversion4/1 -> Demux/1

== system gtm_design/Guidance/CAS Maneuver/High-g Turn ==
  Action Port : ActionPort  ActionPortLabel=case [ 2 ]:
  Bus Creator1 : BusCreator  Inputs=7
  Constant : Constant  Value=alt0
  Constant1 : Constant  Value=tas0
  Constant2 : Constant  Value=0
  Constant3 : Constant  Value=0
  Step : Step  Time=8  Before=10  After=0  SampleTime=0
  Step1 : Step  Time=8  Before=1  After=5  SampleTime=0
  Step2 : Step  Time=8  Before=etas0  After=etas1  SampleTime=0
  Out1 : Outport
  wires:
  Step/1 -> Bus Creator1/6  "p_c_deg"
  Constant/1 -> Bus Creator1/2  "alt_c_ft"
  Bus Creator1/1 -> Out1/1
  Constant2/1 -> Bus Creator1/4  "phi_c_deg"
  Step1/1 -> Bus Creator1/5  "an_c_g"
  Constant3/1 -> Bus Creator1/3  "bet_c_deg"
  Constant1/1 -> Bus Creator1/1  "tas_c_knot"
  Step2/1 -> Bus Creator1/7  "etas_c_percent"

== system gtm_design/Guidance/CAS Maneuver/Label ==
  I : Inport
  Bus Creator1 : BusCreator  Inputs=7
  Demux1 : Demux  Outputs=7
  O : Outport
  wires:
  Bus Creator1/1 -> O/1
  Demux1/4 -> Bus Creator1/4  "phi_c_deg"
  Demux1/2 -> Bus Creator1/2  "alt_c_ft"
  Demux1/6 -> Bus Creator1/6  "p_c_deg"
  Demux1/1 -> Bus Creator1/1  "tas_c_knot"
  Demux1/3 -> Bus Creator1/3  "bet_c_deg"
  Demux1/5 -> Bus Creator1/5  "an_c_g"
  Demux1/7 -> Bus Creator1/7  "etas_c_percent"
  I/1 -> Demux1/1

== system gtm_design/Guidance/CAS Maneuver/Push-over and Pull-up ==
  Action Port : ActionPort  ActionPortLabel=case [ 1 ]:
  Bus Creator1 : BusCreator  Inputs=7
  Constant : Constant  Value=alt0
  Constant1 : Constant  Value=tas0
  Constant2 : Constant  Value=0
  Constant3 : Constant  Value=0
  Constant4 : Constant  Value=0
  Step : Step  Time=5  After=4  SampleTime=0
  Step1 : Step  Time=5  Before=etas0  After=etas1  SampleTime=0
  Out1 : Outport
  wires:
  Constant4/1 -> Bus Creator1/6  "p_c_deg"
  Constant/1 -> Bus Creator1/2  "alt_c_ft"
  Bus Creator1/1 -> Out1/1
  Constant2/1 -> Bus Creator1/4  "phi_c_deg"
  Step/1 -> Bus Creator1/5  "an_c_g"
  Constant3/1 -> Bus Creator1/3  "bet_c_deg"
  Constant1/1 -> Bus Creator1/1  "tas_c_knot"
  Step1/1 -> Bus Creator1/7

== system gtm_design/Guidance/CAS Step/Label ==
  I : Inport
  Bus Creator1 : BusCreator  Inputs=7
  Demux1 : Demux  Outputs=7
  O : Outport
  wires:
  I/1 -> Demux1/1
  Demux1/7 -> Bus Creator1/7  "etas_c_percent"
  Demux1/5 -> Bus Creator1/5  "an_c_g"
  Demux1/3 -> Bus Creator1/3  "bet_c_deg"
  Demux1/1 -> Bus Creator1/1  "tas_c_knot"
  Demux1/6 -> Bus Creator1/6  "p_c_deg"
  Demux1/2 -> Bus Creator1/2  "alt_c_ft"
  Demux1/4 -> Bus Creator1/4  "phi_c_deg"
  Bus Creator1/1 -> O/1

== system gtm_design/Guidance/CAS Step/Normal Acceleration Step Command ==
  Action Port : ActionPort  ActionPortLabel=case [ 1 ]:
  Bus Creator1 : BusCreator  Inputs=7
  Constant : Constant  Value=alt0
  Constant1 : Constant  Value=tas0
  Constant2 : Constant  Value=0
  Constant3 : Constant  Value=0
  Constant4 : Constant  Value=0
  Constant5 : Constant  Value=etas0
  Step : Step  Time=5  After=4  SampleTime=0
  cmd : Outport
  wires:
  Constant1/1 -> Bus Creator1/1  "tas_c_knot"
  Constant3/1 -> Bus Creator1/3  "bet_c_deg"
  Step/1 -> Bus Creator1/5  "an_c_g"
  Constant2/1 -> Bus Creator1/4  "phi_c_deg"
  Bus Creator1/1 -> cmd/1
  Constant/1 -> Bus Creator1/2  "alt_c_ft"
  Constant4/1 -> Bus Creator1/6  "p_c_deg"
  Constant5/1 -> Bus Creator1/7  "etas_c_percent"

== system gtm_design/Guidance/CAS Step/Roll Rate Step Command ==
  Action Port : ActionPort  ActionPortLabel=case [ 3 ]:
  Bus Creator1 : BusCreator  Inputs=7
  Constant : Constant  Value=alt0
  Constant1 : Constant  Value=tas0
  Constant2 : Constant  Value=0
  Constant3 : Constant  Value=0
  Constant4 : Constant
  Constant5 : Constant  Value=etas0
  Step : Step  After=10  SampleTime=0
  cmd : Outport
  wires:
  Constant1/1 -> Bus Creator1/1  "tas_c_knot"
  Constant3/1 -> Bus Creator1/3  "bet_c_deg"
  Constant4/1 -> Bus Creator1/5  "an_c_g"
  Constant2/1 -> Bus Creator1/4  "phi_c_deg"
  Bus Creator1/1 -> cmd/1
  Constant/1 -> Bus Creator1/2  "alt_c_ft"
  Step/1 -> Bus Creator1/6  "p_c_deg"
  Constant5/1 -> Bus Creator1/7  "etas_c_percent"

== system gtm_design/Guidance/CAS Step/Sideslip Step Command ==
  Action Port : ActionPort  ActionPortLabel=case [ 2 ]:
  3deg @ 1sec : Step  After=3  SampleTime=0
  Bus Creator1 : BusCreator  Inputs=7
  Constant : Constant  Value=alt0
  Constant1 : Constant  Value=tas0
  Constant2 : Constant  Value=0
  Constant3 : Constant
  Constant4 : Constant  Value=0
  Constant5 : Constant  Value=etas0
  cmd : Outport
  wires:
  Constant5/1 -> Bus Creator1/7  "etas_c_percent"
  Constant4/1 -> Bus Creator1/6  "p_c_deg"
  Constant/1 -> Bus Creator1/2  "alt_c_ft"
  Bus Creator1/1 -> cmd/1
  Constant2/1 -> Bus Creator1/4  "phi_c_deg"
  Constant3/1 -> Bus Creator1/5  "an_c_g"
  3deg @ 1sec/1 -> Bus Creator1/3  "bet_c_deg"
  Constant1/1 -> Bus Creator1/1  "tas_c_knot"

== system gtm_design/Guidance/CAS Step/Zero ==
  Action Port : ActionPort  ActionPortLabel=default:
  Bus Creator1 : BusCreator  Inputs=7
  Constant : Constant  Value=alt0
  Constant1 : Constant  Value=tas0
  Constant2 : Constant  Value=0
  Constant3 : Constant  Value=0
  Constant4 : Constant  Value=0.9975
  Constant5 : Constant  Value=etas0
  Constant6 : Constant  Value=0
  cmd : Outport
  wires:
  Constant5/1 -> Bus Creator1/7  "etas_c_percent"
  Constant6/1 -> Bus Creator1/6  "p_c_deg"
  Constant/1 -> Bus Creator1/2  "alt_c_ft"
  Bus Creator1/1 -> cmd/1
  Constant2/1 -> Bus Creator1/4  "phi_c_deg"
  Constant4/1 -> Bus Creator1/5  "an_c_g"
  Constant3/1 -> Bus Creator1/3  "bet_c_deg"
  Constant1/1 -> Bus Creator1/1  "tas_c_knot"
